simulink model "GridTiedInverterPortedV3"  (R2025a)
settings: Solver=ode23t  StartTime=0.0  StopTime=0.45  FixedStep=Ts  RelTol=1e-3  EnableMultiTasking=on
PreLoadFcn:
  | GridTiedInverterData;
values from neighbouring files (symbols this model uses):
  Ki_vd = 850    [GridTiedInverterData.m]
  Ki_vq = 850    [GridTiedInverterData.m]
  Kp_vd = 0.36    [GridTiedInverterData.m]
  Kp_vq = 0.36    [GridTiedInverterData.m]
  Ts = 1e-6    (= 1e-06)    [GridTiedInverterData.m]
libraries: nesl_utility x20, fl_lib x15, ee_lib x10, eeTransforms x2, slpidlib x2, eePwmGeneratorTwoLevel x1, eeSinusoidalMeasurement x1
CloseFcn:
  | try,close(h1_GridTiedInverter),end
  | clear h1_GridTiedInverter
  | 
  | 
  | clear simlog_GridTiedInverter
  | clear logsout_GridTiedInverter
  | 
  | clear Ts fsw Kp_vd Ki_vd Kp_vq Ki_vq
Description:
  | Three-Phase Grid-Tied Inverter
settings Model: ExtModeTrigDuration=100  Creator=The MathWorks, Inc.  LastModifiedBy=matthiasmees
settings SolverCC: AlgebraicLoopSolver=TrustRegion  MaxZcPerStep=1.0
settings DataIOCC: SaveFormat=StructureWithTime  SaveOutput=off  SaveTime=off  ReturnWorkspaceOutputs=off  SignalLoggingName=logsout_GridTiedInverter
settings OptimizationCC: ReuseModelBlockBuffer=off  ExpressionDepthLimit=2147483647.0  LifeSpan=inf
settings DebuggingCC: UnconnectedInputMsg=warning  UnconnectedOutputMsg=warning  UnconnectedLineMsg=warning  AllowSymbolicDim=off  StateNameClashWarn=warning  SFUnexpectedBacktrackingDiag=warning  SFNoUnconditionalDefaultTransitionDiag=warning  SFExecutionAtInitializationDiag=none  ArithmeticOperatorsInVariantConditions=warning
settings HardwareCC: ProdBitPerPointer=32.0  ProdBitPerSizeT=32.0  ProdBitPerPtrDiffT=32.0  ProdLargestAtomicFloat=None  ProdIntDivRoundTo=Undefined  ProdEndianess=Unspecified  ProdWordSize=32.0  ProdHWDeviceType=32-bit Generic
settings ModelReferenceCC: EnableRefExpFcnMdlSchedulingChecks=on  PropagateSignalLabelsOutOfModel=off
settings SFSimCC: SimUseLocalCustomCode=off  CustomCodeUndefinedFunction=UseInterfaceOnly
settings RTWCC: RTWUseLocalCustomCode=off  GPUComputeCapability=3.5  DLArmComputeVersion=19.05
settings CodeAppCC: StateflowObjectComments=on
settings GRTTargetCC: TargetLangStandard=C89/C90 (ANSI)  CombineOutputUpdateFcns=off  GRTInterface=on
settings ConfigComp: CovMetricSettings=dw  CovSaveCumulativeToWorkspaceVar=on  CovSaveSingleToWorkspaceVar=on  CovExternalEMLEnable=off
settings SimscapeCC: SimscapeNormalizeSystem=off  SimscapeLogType=all  SimscapeLogName=simlog_GridTiedInverter  SimscapeLogLimitData=off

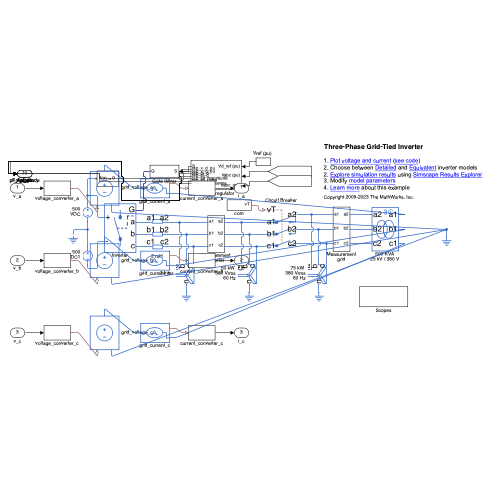
[thumbnail: Simulink's stored preview of the top-level diagram]
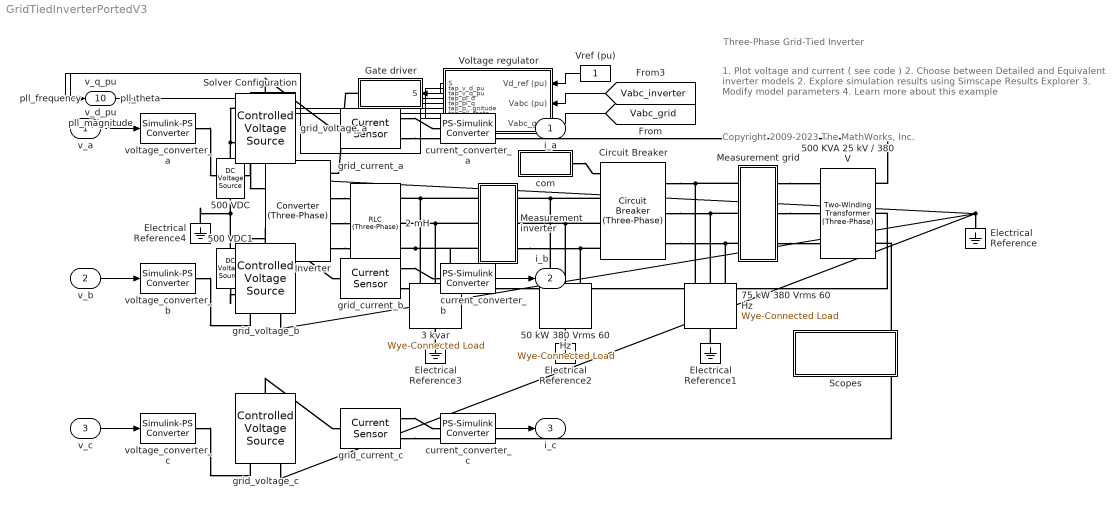
== system GridTiedInverterPortedV3 ==
  note: Three-Phase Grid-Tied Inverter
  note: 1. Plot voltage and current ( see code )
      | 2. Choose between Detailed and Equivalent inverter models
      | 2. Explore simulation results using Simscape Results Explorer
      | 3. Modify model parameters
      | 4. Learn more about this example
  note: Copyright 2009-2023 The MathWorks, Inc.
  v_a : Inport
  v_b : Inport  Port=2
  v_c : Inport  Port=3
  2 mH : ee_lib/Passive/RLC Assemblies/RLC (Three-Phase)  port_option=ee.enum.threePhasePort.expanded  component_structure=ee.enum.rlc.structure.SeriesRL  R=0.02 Ohm  L=0.002 H  C=1 F  R_parasitic=1e-6 Ohm  G_parasitic=1e-6 1/Ohm  IL_specify=on  IL_priority=High  IL=[0, 0, 0] A  IL_nominal_specify=off  IL_nominal_value=1  IL_nominal_unit=A  VC_specify=on  VC_priority=High  VC=[0, 0, 0] V  VC_nominal_specify=off  VC_nominal_value=1  VC_nominal_unit=V
      settings: InternalSimscapePortConfiguration="{\"Bottom\":[],\"Left\":[{\"id\":\"a1\",\"label\":\"a1\",\"type\":\"foundation.electrical.electrical\"},{\"id\":\"b1\",\"label\":\"b1\",\"type\":\"foundation.electrical.electrical\"},{\"id\":\"c1\",\"label\":\"c1\",\"type\":\"foundation.electrical.electrical\"}],\"Right\":[{\"id\":\"a2\",\"label\":\"a2\",\"type\":\"foundation.electrical.electrical\"},{\"id\":\"b2\",\"label\":\"b2\",\"type\":\"foundation.electrical.electrical\"},{\"id\":\"c2\",\"label\":\"c2\",\"type\":\"foundation.electrical.electrical\"}],\"Top\":[]}"
  3 kvar : ee_lib/Passive/RLC Assemblies/Wye-Connected Load  port_option=ee.enum.threePhasePort.expanded  parameterization=ee.enum.rlc.parameterization.ratedpower  component_structure=ee.enum.rlc.structure.C  component_structure_PQ=ee.enum.rlc.structure.C  R=1 Ohm  L=0.001 H  C=1e-6 F  VRated=380 V  FRated=60 Hz  P=0 W  Qpos=0 V*A  Qneg=-3000 V*A  R_parasitic=1e-6 Ohm  G_parasitic=1e-6 1/Ohm  R_parasitic_PQ=1e-6 Ohm  G_parasitic_PQ=1e-6 1/Ohm  Vmag0=0 V  Vang0=0 deg  Freq0=60 Hz  IL_specify=on  IL_priority=High  IL=[ 0 0 0 ] A  IL_nominal_specify=off  IL_nominal_value=1  IL_nominal_unit=A  VC_specify=on  VC_priority=High  VC=[ 0 0 0 ] V  VC_nominal_specify=off  VC_nominal_value=1  VC_nominal_unit=V
      settings: InternalSimscapePortConfiguration="{\"Bottom\":[],\"Left\":[{\"id\":\"a\",\"label\":\"a\",\"type\":\"foundation.electrical.electrical\"},{\"id\":\"b\",\"label\":\"b\",\"type\":\"foundation.electrical.electrical\"},{\"id\":\"c\",\"label\":\"c\",\"type\":\"foundation.electrical.electrical\"}],\"Right\":[{\"id\":\"n\",\"label\":\"n\",\"type\":\"foundation.electrical.electrical\"}],\"Top\":[]}"
  50 kW 380 Vrms 60 Hz : ee_lib/Passive/RLC Assemblies/Wye-Connected Load  port_option=ee.enum.threePhasePort.expanded  parameterization=2  component_structure=1  component_structure_PQ=ee.enum.rlc.structure.R  R=1 Ohm  L=0.001 H  C=1e-6 F  VRated=380 V  FRated=60 Hz  P=50000 W  Qpos=0 V*A  Qneg=-3000 V*A  R_parasitic=1e-6 Ohm  G_parasitic=1e-6 1/Ohm  R_parasitic_PQ=1e-6 Ohm  G_parasitic_PQ=1e-6 1/Ohm  Vmag0=380 V  Vang0=0 deg  Freq0=60 Hz  IL_specify=on  IL_priority=High  IL=[ 0 0 0 ] A  IL_nominal_specify=off  IL_nominal_value=1  IL_nominal_unit=A  VC_specify=on  VC_priority=High  VC=[ 0 0 0 ] V  VC_nominal_specify=off  VC_nominal_value=1  VC_nominal_unit=V
      settings: InternalSimscapePortConfiguration="{\"Bottom\":[],\"Left\":[{\"id\":\"a\",\"label\":\"a\",\"type\":\"foundation.electrical.electrical\"},{\"id\":\"b\",\"label\":\"b\",\"type\":\"foundation.electrical.electrical\"},{\"id\":\"c\",\"label\":\"c\",\"type\":\"foundation.electrical.electrical\"}],\"Right\":[{\"id\":\"n\",\"label\":\"n\",\"type\":\"foundation.electrical.electrical\"}],\"Top\":[]}"
  500 VDC : fl_lib/Electrical/Electrical Sources/DC Voltage Source  v0=500 V
  500 VDC1 : fl_lib/Electrical/Electrical Sources/DC Voltage Source  v0=500 V
  500 KVA 25 kV / 380 V : ee_lib/Passive/Transformers/Two-Winding Transformer (Three-Phase)  SRated=500000 V*A  FRated=60 Hz  Winding1Connection=ee.enum.windingconnection.Y  VRated1=25000 V  Winding2Connection=ee.enum.windingconnection.delta1  VRated2=380 V  CoreType=ee.enum.coretype.fivelimb  pu_Rw1=0.0020  pu_Rw2=0.0020  leakage_reactance_option=ee.enum.transformer_leakage.include  pu_Xl1=0.0800  pu_Xl2=0.0800  magnetizing_resistance_option=ee.enum.transformer_magnetizingResistance.include  pu_Rm=500  magnetizing_reactance_option=ee.enum.transformer_magnetizingReactance.include  saturation_option=ee.enum.transformer_saturation.exclude  pu_Xm=500  current_data=[0, .002, 1, 2]  magnetic_flux_data=[0, 1.2, 1.5, 1.51]  pu_X0=0.5  i1_specify=off  i1_priority=None  i1=[ 0 0 0 ] A  i1_nominal_specify=off  i1_nominal_value=1  i1_nominal_unit=A  i2_specify=off  i2_priority=None  i2=[ 0 0 0 ] A  i2_nominal_specify=off  i2_nominal_value=1  i2_nominal_unit=A  phi_specify=on  phi_priority=None  phi=[0, 0, 0]  phi_nominal_specify=off  phi_nominal_value=1  phi_nominal_unit=1  power_dissipated_specify=off  power_dissipated_priority=None  power_dissipated=0 W  power_dissipated_nominal_specify=off  power_dissipated_nominal_value=1  power_dissipated_nominal_unit=W
      settings: InternalSimscapePortConfiguration="{\"Bottom\":[],\"Left\":[{\"id\":\"a1\",\"label\":\"a1\",\"type\":\"foundation.electrical.electrical\"},{\"id\":\"b1\",\"label\":\"b1\",\"type\":\"foundation.electrical.electrical\"},{\"id\":\"c1\",\"label\":\"c1\",\"type\":\"foundation.electrical.electrical\"}],\"Right\":[{\"id\":\"a2\",\"label\":\"a2\",\"type\":\"foundation.electrical.electrical\"},{\"id\":\"b2\",\"label\":\"b2\",\"type\":\"foundation.electrical.electrical\"},{\"id\":\"c2\",\"label\":\"c2\",\"type\":\"foundation.electrical.electrical\"}],\"Top\":[]}"
  75 kW 380 Vrms 60 Hz : ee_lib/Passive/RLC Assemblies/Wye-Connected Load  port_option=ee.enum.threePhasePort.expanded  parameterization=2  component_structure=1  component_structure_PQ=ee.enum.rlc.structure.R  R=1 Ohm  L=0.001 H  C=1e-6 F  VRated=380 V  FRated=60 Hz  P=75000 W  Qpos=0 V*A  Qneg=-3000 V*A  R_parasitic=1e-6 Ohm  G_parasitic=1e-6 1/Ohm  R_parasitic_PQ=1e-6 Ohm  G_parasitic_PQ=1e-6 1/Ohm  Vmag0=380 V  Vang0=0 deg  Freq0=60 Hz  IL_specify=on  IL_priority=High  IL=[ 0 0 0 ] A  IL_nominal_specify=off  IL_nominal_value=1  IL_nominal_unit=A  VC_specify=on  VC_priority=High  VC=[ 0 0 0 ] V  VC_nominal_specify=off  VC_nominal_value=1  VC_nominal_unit=V
      settings: InternalSimscapePortConfiguration="{\"Bottom\":[],\"Left\":[{\"id\":\"a\",\"label\":\"a\",\"type\":\"foundation.electrical.electrical\"},{\"id\":\"b\",\"label\":\"b\",\"type\":\"foundation.electrical.electrical\"},{\"id\":\"c\",\"label\":\"c\",\"type\":\"foundation.electrical.electrical\"}],\"Right\":[{\"id\":\"n\",\"label\":\"n\",\"type\":\"foundation.electrical.electrical\"}],\"Top\":[]}"
  Circuit Breaker : ee_lib/Switches & Breakers/Circuit Breaker (Three-Phase)  R_closed=0.001 Ohm  G_open=1e-6 1/Ohm  threshold=0.5 V  breaker_behavior=ee.enum.switches.breakerBehavior.zeroCrossingEnable
      settings: InternalSimscapePortConfiguration="{\"Bottom\":[],\"Left\":[{\"id\":\"vT\",\"label\":\"vT\",\"type\":\"input\"},{\"id\":\"a1\",\"label\":\"a1\",\"type\":\"foundation.electrical.electrical\"},{\"id\":\"b1\",\"label\":\"b1\",\"type\":\"foundation.electrical.electrical\"},{\"id\":\"c1\",\"label\":\"c1\",\"type\":\"foundation.electrical.electrical\"}],\"Right\":[{\"id\":\"a2\",\"label\":\"a2\",\"type\":\"foundation.electrical.electrical\"},{\"id\":\"b2\",\"label\":\"b2\",\"type\":\"foundation.electrical.electrical\"},{\"id\":\"c2\",\"label\":\"c2\",\"type\":\"foundation.electrical.electrical\"}],\"Top\":[]}"
  Electrical Reference{,1..4} (5 alike) : fl_lib/Electrical/Electrical Elements/Electrical Reference
  Gate driver : Subsystem
  Inverter : ee_lib/Semiconductors & Converters/Converters/Converter (Three-Phase)  port_option=ee.enum.threePhasePort.expanded  fidelity_option=ee.enum.converters.fidelity.detailed  device_type=ee.enum.converters.switchingdevice.igbt  showThermalPort=false  K=0  Vth=0.5 V  Vgt=0.5 V  Vgt_off=0.1 V  Ih=0.1 A  Vf=1e-6 V  Ron=1e-3 Ohm  Rds=0.001 Ohm  Goff=2e-4 1/Ohm  Eon_scalar=22.86e-3 J  Eoff_scalar=17.14e-3 J  Eoff_natural_commutation=10e-3 J  Voff=300 V  Iout_scalar=600 A  onCurrentMeasDelay=0 s  useCurrentFromPreviousCycle=false  useVoltageFromPreviousCycle=false  diode_param=ee.enum.converters.protectiondiode.nodynamics  diode_Vf=1e-6 V  diode_Ron=1e-3 Ohm  diode_Goff=2e-4 1/Ohm  diode_C=50 nF  diode_iRM=-235 A  diode_iF=300 A  diode_idot=-50 A/us  diode_trr_param=ee.enum.converters.diodetrr.trr_factor  diode_trr_factor=3  diode_trr=15 us  diode_Qrr=1.5e+3 s*uA  diode_rec_loss_model=ee.enum.diode.reverseRecoveryModel.fixed  diode_ErecVal=0 J  diode_scaleWithIandV=false  diode_ErecMat=zeros(2, 3) J  diode_TjrecVec=[298.15, 398.15] K  diode_IfrecVec=[.1, 1, 10] A  diode_IrecVal=10 A  diode_VrecVal=10 V  diode_tFilter=1 / 1000 / 100 s  thermal_network_parameterization=ee.enum.thermalNetworkTopology.external  Rth=[.08, .5] K/W  Rth_Cauer=[.08, .1, .5] K/W  Rth_Foster=[.08, .14, .22, .16] K/W  thermal_mass_parameterization=ee.enum.thermalNetwork.timeconstant  thermal_mass=[.01, .5] J/K  thermal_mass_Cauer=[.01, .1, .5] J/K  thermal_mass_Foster=[.001, .005, .05, .5] J/K  thermal_time_constant=[.001, .2] s  thermal_time_constant_Cauer=[.001, .1, .2] s  thermal_time_constant_Foster=[7e-05, .0007, .01, .08] s  thermal_mass_initial_temperatures=[25, 25] degC  thermal_mass_initial_temperatures_Cauer=[25, 25, 25] degC  junction_thermal_mass=0.01 J/K  Tvec_initial_Foster=[25, 25, 25, 25] degC  snubber_type=ee.enum.converters.snubber.exclude  Cs=1e-7 F  Rs=0.1 Ohm  Vce_loss=[0, 150, 300] V
      settings: InternalSimscapePortConfiguration="{\"Bottom\":[],\"Left\":[{\"id\":\"G\",\"label\":\"G\",\"type\":\"foundation.electrical.twelve_phase\"},{\"id\":\"a\",\"label\":\"a\",\"type\":\"foundation.electrical.electrical\"},{\"id\":\"b\",\"label\":\"b\",\"type\":\"foundation.electrical.electrical\"},{\"id\":\"c\",\"label\":\"c\",\"type\":\"foundation.electrical.electrical\"}],\"Right\":[{\"id\":\"p\",\"label\":\"+\",\"type\":\"foundation.electrical.electrical\"},{\"id\":\"n\",\"label\":\"-\",\"type\":\"foundation.electrical.electrical\"}],\"Top\":[]}"
  Measurement grid : Subsystem
  Measurement inverter : Subsystem
  Scopes : Subsystem
  Solver Configuration : nesl_utility/Solver Configuration  PhysicalDomain=network_engine_domain  SubClassName=solver  LeftPortType=input  RightPortType=generic  Tones=[]  Harmonics=[]  SimulateNoise=off  Profile=off  UseLocalSampling=off  EnableSwitchedLinearOptims=on  FrequencyDomain=off  UseCCode=off  RelTol=0.001  AbsTol=1e-06  MinStep=1e-09  ToWorkspace=off  RevertToSquareIcSolve=off  NumHomotopyIterations=100  PhasorMode=off  PhasorModeNumHarmonics=1  ConsistencySolver=NEWTON_FTOL  IndexReductionMethod=DerivativeReplacement  DoDC=off  ResidualTolerance=1e-09  ConsistencyTolSource=GLOBAL  ConsistencyAbsTol=0.001  ConsistencyRelTol=0.001  ConsistencyTolFactor=0.001  UseLocalSolver=off  LocalSolverChoice=NE_BACKWARD_EULER_ADVANCER  ResolveIndetEquations=on  FunctionEvalNumThread=1  LocalSolverSampleTime=Ts  DoFixedCost=off  MaxNonlinIter=3  MaxModeIter=2  ComputeImpulses=off  ImpulseIterations=1  LinearAlgebra=auto  LinearAlgebraNumThread=0  EquationFormulation=NE_TIME_EF  DelaysMemoryBudget=1024  AutomaticFiltering=on  FilteringTimeConstant=0.001  PartitionStorageMethod=AS_NEEDED  PartitionMemoryBudget=1024  PartitionMethod=FAST  MultibodyUseLocalSolver=off  MultibodyLocalSolverChoice=ODE1  MultibodyLocalSolverSampleTime=0.001
  Voltage regulator : Subsystem
  "Vref (pu) " : Constant
  com : Subsystem
  current_converter_a : nesl_utility/PS-Simulink Converter  PhysicalDomain=network_engine_domain  SubClassName=ps_output  LeftPortType=input  RightPortType=output  PseudoPeriodic=off  Frequencies=[]  VectorFormat=inherit  Unit=A  AffineConversion=off
  current_converter_b : nesl_utility/PS-Simulink Converter  PhysicalDomain=network_engine_domain  SubClassName=ps_output  LeftPortType=input  RightPortType=output  PseudoPeriodic=off  Frequencies=[]  VectorFormat=inherit  Unit=A  AffineConversion=off
  current_converter_c : nesl_utility/PS-Simulink Converter  PhysicalDomain=network_engine_domain  SubClassName=ps_output  LeftPortType=input  RightPortType=output  PseudoPeriodic=off  Frequencies=[]  VectorFormat=inherit  Unit=A  AffineConversion=off
  grid_current_a : fl_lib/Electrical/Electrical Sensors/Current Sensor
  grid_current_b : fl_lib/Electrical/Electrical Sensors/Current Sensor
  grid_current_c : fl_lib/Electrical/Electrical Sensors/Current Sensor
  grid_voltage_a : fl_lib/Electrical/Electrical Sources/Controlled Voltage Source
  grid_voltage_b : fl_lib/Electrical/Electrical Sources/Controlled Voltage Source
  grid_voltage_c : fl_lib/Electrical/Electrical Sources/Controlled Voltage Source
  voltage_converter_a : nesl_utility/Simulink-PS Converter  PhysicalDomain=network_engine_domain  SubClassName=ps_input  LeftPortType=input  RightPortType=output  PseudoPeriodic=off  Frequencies=[]  NoiseDistribution=none  NoiseParameters=[]  Unit=V  AffineConversion=off  FilteringAndDerivatives=provide  SimscapeFilterOrder=1  InputFilterTimeConstant=0.001  UdotUserProvided=0
  voltage_converter_b : nesl_utility/Simulink-PS Converter  PhysicalDomain=network_engine_domain  SubClassName=ps_input  LeftPortType=input  RightPortType=output  PseudoPeriodic=off  Frequencies=[]  NoiseDistribution=none  NoiseParameters=[]  Unit=V  AffineConversion=off  FilteringAndDerivatives=provide  SimscapeFilterOrder=1  InputFilterTimeConstant=0.001  UdotUserProvided=0
  voltage_converter_c : nesl_utility/Simulink-PS Converter  PhysicalDomain=network_engine_domain  SubClassName=ps_input  LeftPortType=input  RightPortType=output  PseudoPeriodic=off  Frequencies=[]  NoiseDistribution=none  NoiseParameters=[]  Unit=V  AffineConversion=off  FilteringAndDerivatives=provide  SimscapeFilterOrder=1  InputFilterTimeConstant=0.001  UdotUserProvided=0
  i_a : Outport
  i_b : Outport  Port=2
  i_c : Outport  Port=3
  v_d_pu : Outport  Port=4
  v_q_pu : Outport  Port=5
  pi_d : Outport  Port=6
  pi_q : Outport  Port=7
  pll_frequency : Outport  Port=8
  pll_theta : Outport  Port=9
  pll_magnitude : Outport  Port=10
  wires:
  [Vabc_grid] -> Voltage regulator/3(Vabc_grid)
  "Vref (pu) "/1 -> Voltage regulator/1(Vd_ref (pu))
  [Vabc_inverter] -> Voltage regulator/2(Vabc (pu))
  Voltage regulator/1(S) -> Gate driver/1(S)
  v_a/1 -> voltage_converter_a/1
  current_converter_a/1 -> i_a/1
  v_b/1 -> voltage_converter_b/1
  current_converter_b/1 -> i_b/1
  v_c/1 -> voltage_converter_c/1
  current_converter_c/1 -> i_c/1
  Voltage regulator/2(tap_v_d_pu) -> v_d_pu/1
  Voltage regulator/3(tap_v_q_pu) -> v_q_pu/1
  Voltage regulator/4(tap_pi_d) -> pi_d/1
  Voltage regulator/5(tap_pi_q) -> pi_q/1
  Voltage regulator/6(tap_pll_magnitude) -> pll_frequency/1
  Voltage regulator/7(tap_pll_theta) -> pll_theta/1
  Voltage regulator/8(tap_pll_frequency) -> pll_magnitude/1
  connections:
  75 kW 380 Vrms 60 Hz/LConn1 -- Measurement grid/LConn1 -- Circuit Breaker/RConn1
  3 kvar/LConn2 -- Measurement inverter/LConn2 -- 2 mH/RConn2
  Circuit Breaker/LConn2 -- 50 kW 380 Vrms 60 Hz/LConn1 -- Measurement inverter/RConn1
  Circuit Breaker/RConn2 -- Measurement grid/LConn2 -- 75 kW 380 Vrms 60 Hz/LConn2
  Measurement grid/RConn3 -- 500 KVA 25 kV / 380 V/RConn3
  500 VDC/LConn1 -- Solver Configuration/RConn1 -- Inverter/RConn1
  Circuit Breaker/RConn3 -- Measurement grid/LConn3 -- 75 kW 380 Vrms 60 Hz/LConn3
  50 kW 380 Vrms 60 Hz/LConn3 -- Circuit Breaker/LConn4 -- Measurement inverter/RConn3
  Inverter/LConn4 -- 2 mH/LConn3
  Electrical Reference1/LConn1 -- 75 kW 380 Vrms 60 Hz/RConn1
  Gate driver/RConn1 -- Inverter/LConn1
  Electrical Reference2/LConn1 -- 50 kW 380 Vrms 60 Hz/RConn1
  com/RConn1 -- Circuit Breaker/LConn1
  Electrical Reference3/LConn1 -- 3 kvar/RConn1
  Inverter/LConn2 -- 2 mH/LConn1
  Inverter/LConn3 -- 2 mH/LConn2
  3 kvar/LConn1 -- 2 mH/RConn1 -- Measurement inverter/LConn1
  2 mH/RConn3 -- Measurement inverter/LConn3 -- 3 kvar/LConn3
  Circuit Breaker/LConn3 -- 50 kW 380 Vrms 60 Hz/LConn2 -- Measurement inverter/RConn2
  Measurement grid/RConn1 -- 500 KVA 25 kV / 380 V/RConn1
  Measurement grid/RConn2 -- 500 KVA 25 kV / 380 V/RConn2
  500 VDC1/RConn1 -- Inverter/RConn2
  500 VDC1/LConn1 -- Electrical Reference4/LConn1 -- 500 VDC/RConn1
  voltage_converter_a/RConn1 -- grid_voltage_a/RConn1
  grid_voltage_a/LConn1 -- grid_current_a/LConn1
  grid_current_a/RConn2 -- 500 KVA 25 kV / 380 V/LConn1
  grid_current_a/RConn1 -- current_converter_a/LConn1
  voltage_converter_b/RConn1 -- grid_voltage_b/RConn1
  grid_voltage_b/LConn1 -- grid_current_b/LConn1
  grid_current_b/RConn2 -- 500 KVA 25 kV / 380 V/LConn2
  grid_current_b/RConn1 -- current_converter_b/LConn1
  voltage_converter_c/RConn1 -- grid_voltage_c/RConn1
  grid_voltage_c/LConn1 -- grid_current_c/LConn1
  grid_current_c/RConn2 -- 500 KVA 25 kV / 380 V/LConn3
  grid_current_c/RConn1 -- current_converter_c/LConn1
  grid_voltage_a/RConn2 -- grid_voltage_b/RConn2 -- Electrical Reference/LConn1 -- grid_voltage_c/RConn2

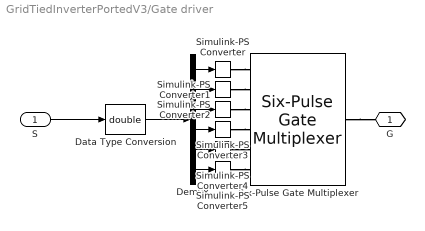
== system GridTiedInverterPortedV3/Gate driver ==
  S : Inport
  Data Type Conversion : DataTypeConversion  OutDataTypeStr=double  SaturateOnIntegerOverflow=off  RndMeth=Floor
  Demux : Demux  Outputs=6
  Simulink-PS Converter{,1..5} (6 alike) : nesl_utility/Simulink-PS Converter  PhysicalDomain=network_engine_domain  SubClassName=ps_input  LeftPortType=input  RightPortType=output  PseudoPeriodic=off  Frequencies=[]  NoiseDistribution=none  NoiseParameters=[]  Unit=1  AffineConversion=off  FilteringAndDerivatives=provide  SimscapeFilterOrder=1  InputFilterTimeConstant=0.001  UdotUserProvided=0
  Six-Pulse Gate Multiplexer : ee_lib/Semiconductors & Converters/Converters/Six-Pulse Gate Multiplexer  port_option=ee.enum.controlport.ps
  G : PMIOPort  Side=Right
  wires:
  Demux/5 -> Simulink-PS Converter4/1
  Demux/3 -> Simulink-PS Converter2/1
  Data Type Conversion/1 -> Demux/1
  Demux/4 -> Simulink-PS Converter3/1
  Demux/6 -> Simulink-PS Converter5/1
  Demux/2 -> Simulink-PS Converter1/1
  Demux/1 -> Simulink-PS Converter/1
  S/1 -> Data Type Conversion/1
  connections:
  Simulink-PS Converter4/RConn1 -- Six-Pulse Gate Multiplexer/LConn5
  Simulink-PS Converter2/RConn1 -- Six-Pulse Gate Multiplexer/LConn3
  Simulink-PS Converter/RConn1 -- Six-Pulse Gate Multiplexer/LConn1
  Simulink-PS Converter5/RConn1 -- Six-Pulse Gate Multiplexer/LConn6
  Simulink-PS Converter1/RConn1 -- Six-Pulse Gate Multiplexer/LConn2
  Simulink-PS Converter3/RConn1 -- Six-Pulse Gate Multiplexer/LConn4
  Six-Pulse Gate Multiplexer/RConn1 -- G/RConn1

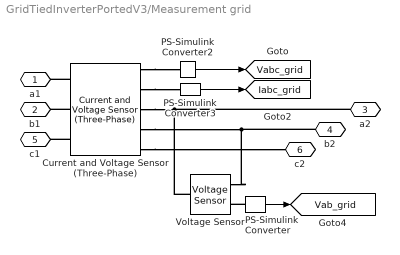
== system GridTiedInverterPortedV3/Measurement grid ==
  Current and Voltage Sensor (Three-Phase) : ee_lib/Sensors & Transducers/Current and Voltage Sensor (Three-Phase)  vMeasurementType=2  outputUnit=ee.enum.unit.pu  SRated=250000 V*A  VRated=380 V  I_specify=off  I_priority=None  I=[ 0 0 0 ] A  I_nominal_specify=off  I_nominal_value=1  I_nominal_unit=A  V_specify=off  V_priority=None  V=[ 0 0 0 ] V  V_nominal_specify=off  V_nominal_value=1  V_nominal_unit=V
      settings: InternalSimscapePortConfiguration="{\"Bottom\":[],\"Left\":[{\"id\":\"a1\",\"label\":\"a1\",\"type\":\"foundation.electrical.electrical\"},{\"id\":\"b1\",\"label\":\"b1\",\"type\":\"foundation.electrical.electrical\"},{\"id\":\"c1\",\"label\":\"c1\",\"type\":\"foundation.electrical.electrical\"}],\"Right\":[{\"id\":\"V_output\",\"label\":\"V\",\"type\":\"output\"},{\"id\":\"I_output\",\"label\":\"I\",\"type\":\"output\"},{\"id\":\"a2\",\"label\":\"a2\",\"type\":\"foundation.electrical.electrical\"},{\"id\":\"b2\",\"label\":\"b2\",\"type\":\"foundation.electrical.electrical\"},{\"id\":\"c2\",\"label\":\"c2\",\"type\":\"foundation.electrical.electrical\"}],\"Top\":[]}"
  PS-Simulink Converter : nesl_utility/PS-Simulink Converter  PhysicalDomain=network_engine_domain  SubClassName=ps_output  LeftPortType=input  RightPortType=output  PseudoPeriodic=off  Frequencies=[]  VectorFormat=1-D array  Unit=V  AffineConversion=off
  PS-Simulink Converter2 : nesl_utility/PS-Simulink Converter  PhysicalDomain=network_engine_domain  SubClassName=ps_output  LeftPortType=input  RightPortType=output  PseudoPeriodic=off  Frequencies=[]  VectorFormat=1-D array  Unit=1  AffineConversion=off
  PS-Simulink Converter3 : nesl_utility/PS-Simulink Converter  PhysicalDomain=network_engine_domain  SubClassName=ps_output  LeftPortType=input  RightPortType=output  PseudoPeriodic=off  Frequencies=[]  VectorFormat=1-D array  Unit=1  AffineConversion=off
  Voltage Sensor : fl_lib/Electrical/Electrical Sensors/Voltage Sensor
  a1 : PMIOPort  Side=Left
  b1 : PMIOPort  Port=2  Side=Left
  a2 : PMIOPort  Port=3  Side=Right
  b2 : PMIOPort  Port=4  Side=Right
  c1 : PMIOPort  Port=5  Side=Left
  c2 : PMIOPort  Port=6  Side=Right
  tag scope: Iabc_grid=global, Vab_grid=global, Vabc_grid=global
  wires:
  PS-Simulink Converter2/1 -> [Vabc_grid]
  PS-Simulink Converter3/1 -> [Iabc_grid]
  PS-Simulink Converter/1 -> [Vab_grid]
  connections:
  b2/RConn1 -- Voltage Sensor/RConn2 -- Current and Voltage Sensor (Three-Phase)/RConn4
  a2/RConn1 -- Voltage Sensor/LConn1 -- Current and Voltage Sensor (Three-Phase)/RConn3
  Current and Voltage Sensor (Three-Phase)/RConn5 -- c2/RConn1
  Current and Voltage Sensor (Three-Phase)/LConn2 -- b1/RConn1
  Current and Voltage Sensor (Three-Phase)/LConn3 -- c1/RConn1
  Current and Voltage Sensor (Three-Phase)/LConn1 -- a1/RConn1
  Current and Voltage Sensor (Three-Phase)/RConn1 -- PS-Simulink Converter2/LConn1
  Current and Voltage Sensor (Three-Phase)/RConn2 -- PS-Simulink Converter3/LConn1
  PS-Simulink Converter/LConn1 -- Voltage Sensor/RConn1

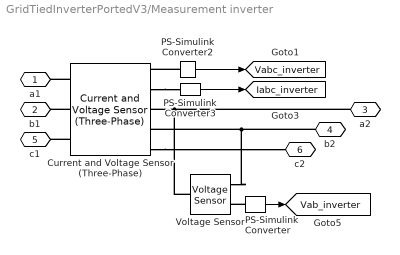
== system GridTiedInverterPortedV3/Measurement inverter ==
  Current and Voltage Sensor (Three-Phase) : ee_lib/Sensors & Transducers/Current and Voltage Sensor (Three-Phase)  vMeasurementType=2  outputUnit=1  SRated=150000 V*A  VRated=380 V  I_specify=off  I_priority=None  I=[ 0 0 0 ] A  I_nominal_specify=off  I_nominal_value=1  I_nominal_unit=A  V_specify=off  V_priority=None  V=[ 0 0 0 ] V  V_nominal_specify=off  V_nominal_value=1  V_nominal_unit=V
      settings: InternalSimscapePortConfiguration="{\"Bottom\":[],\"Left\":[{\"id\":\"a1\",\"label\":\"a1\",\"type\":\"foundation.electrical.electrical\"},{\"id\":\"b1\",\"label\":\"b1\",\"type\":\"foundation.electrical.electrical\"},{\"id\":\"c1\",\"label\":\"c1\",\"type\":\"foundation.electrical.electrical\"}],\"Right\":[{\"id\":\"V_output\",\"label\":\"V\",\"type\":\"output\"},{\"id\":\"I_output\",\"label\":\"I\",\"type\":\"output\"},{\"id\":\"a2\",\"label\":\"a2\",\"type\":\"foundation.electrical.electrical\"},{\"id\":\"b2\",\"label\":\"b2\",\"type\":\"foundation.electrical.electrical\"},{\"id\":\"c2\",\"label\":\"c2\",\"type\":\"foundation.electrical.electrical\"}],\"Top\":[]}"
  PS-Simulink Converter : nesl_utility/PS-Simulink Converter  PhysicalDomain=network_engine_domain  SubClassName=ps_output  LeftPortType=input  RightPortType=output  PseudoPeriodic=off  Frequencies=[]  VectorFormat=1-D array  Unit=V  AffineConversion=off
  PS-Simulink Converter2 : nesl_utility/PS-Simulink Converter  PhysicalDomain=network_engine_domain  SubClassName=ps_output  LeftPortType=input  RightPortType=output  PseudoPeriodic=off  Frequencies=[]  VectorFormat=1-D array  Unit=1  AffineConversion=off
  PS-Simulink Converter3 : nesl_utility/PS-Simulink Converter  PhysicalDomain=network_engine_domain  SubClassName=ps_output  LeftPortType=input  RightPortType=output  PseudoPeriodic=off  Frequencies=[]  VectorFormat=1-D array  Unit=1  AffineConversion=off
  Voltage Sensor : fl_lib/Electrical/Electrical Sensors/Voltage Sensor
  a1 : PMIOPort  Side=Left
  b1 : PMIOPort  Port=2  Side=Left
  a2 : PMIOPort  Port=3  Side=Right
  b2 : PMIOPort  Port=4  Side=Right
  c1 : PMIOPort  Port=5  Side=Left
  c2 : PMIOPort  Port=6  Side=Right
  tag scope: Iabc_inverter=global, Vab_inverter=global, Vabc_inverter=global
  wires:
  PS-Simulink Converter2/1 -> [Vabc_inverter]
  PS-Simulink Converter3/1 -> [Iabc_inverter]
  PS-Simulink Converter/1 -> [Vab_inverter]
  connections:
  b2/RConn1 -- Voltage Sensor/RConn2 -- Current and Voltage Sensor (Three-Phase)/RConn4
  a2/RConn1 -- Voltage Sensor/LConn1 -- Current and Voltage Sensor (Three-Phase)/RConn3
  Current and Voltage Sensor (Three-Phase)/RConn5 -- c2/RConn1
  Current and Voltage Sensor (Three-Phase)/LConn2 -- b1/RConn1
  Current and Voltage Sensor (Three-Phase)/LConn3 -- c1/RConn1
  Current and Voltage Sensor (Three-Phase)/LConn1 -- a1/RConn1
  PS-Simulink Converter2/LConn1 -- Current and Voltage Sensor (Three-Phase)/RConn1
  Current and Voltage Sensor (Three-Phase)/RConn2 -- PS-Simulink Converter3/LConn1
  PS-Simulink Converter/LConn1 -- Voltage Sensor/RConn1

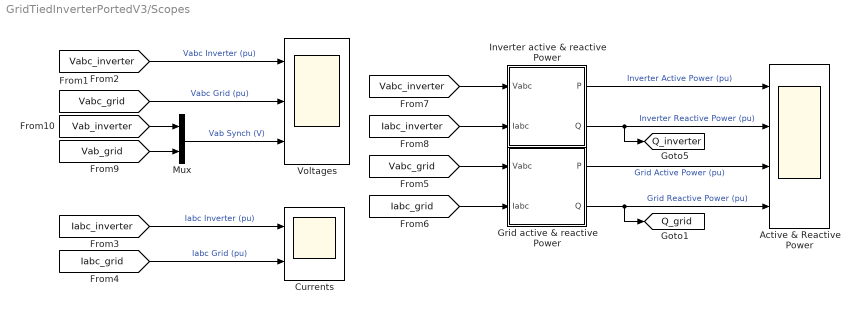
== system GridTiedInverterPortedV3/Scopes ==
  Active & Reactive Power : Scope  NumInputPorts=4
      settings: ActiveDisplayYMinimum=-0.09819  ActiveDisplayYMaximum=0.88371  DataLoggingDecimation=10
  Currents : Scope  NumInputPorts=2
      settings: ActiveDisplayYMinimum=-0.75017  ActiveDisplayYMaximum=0.74928  DataLoggingVariableName=ScopeData2
  Grid active & reactive Power : Subsystem
  "Inverter active & reactive Power " : Subsystem
  Mux : Mux  Inputs=2
  Voltages : Scope  NumInputPorts=3
      settings: ActiveDisplayYMinimum=-1.26809  ActiveDisplayYMaximum=1.26724
  tag scope: Q_grid=global, Q_inverter=global
  wires:
  [Iabc_grid] -> Grid active & reactive Power/2(Iabc)
  "Inverter active & reactive Power "/2(Q) -> Active & Reactive Power/2, [Q_inverter]  "Inverter Reactive Power (pu)"
  [Vab_grid] -> Mux/2
  [Vab_inverter] -> Mux/1
  [Iabc_inverter] -> Currents/1  "Iabc Inverter (pu)"
  Mux/1 -> Voltages/3  "Vab Synch (V)"
  [Vabc_inverter] -> Voltages/1  "Vabc Inverter (pu)"
  [Iabc_inverter] -> "Inverter active & reactive Power "/2(Iabc)
  [Vabc_grid] -> Grid active & reactive Power/1(Vabc)
  [Vabc_inverter] -> "Inverter active & reactive Power "/1(Vabc)
  [Iabc_grid] -> Currents/2  "Iabc Grid (pu)"
  [Vabc_grid] -> Voltages/2  "Vabc Grid (pu)"
  Grid active & reactive Power/2(Q) -> [Q_grid], Active & Reactive Power/4  "Grid Reactive Power (pu)"
  "Inverter active & reactive Power "/1(P) -> Active & Reactive Power/1  "Inverter Active Power (pu)"
  Grid active & reactive Power/1(P) -> Active & Reactive Power/3  "Grid Active Power (pu)"

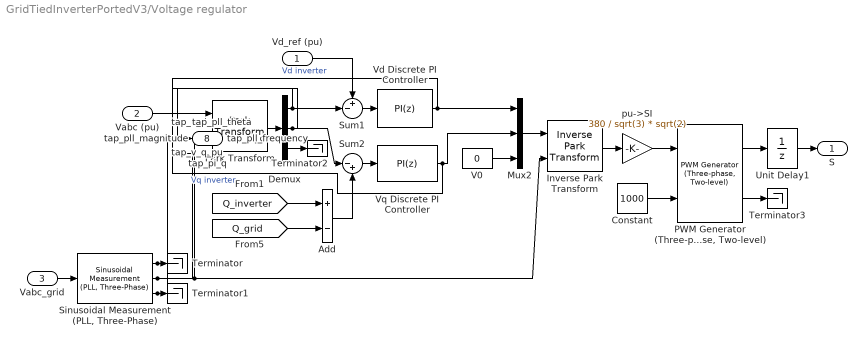
== system GridTiedInverterPortedV3/Voltage regulator ==
  Vd_ref (pu) : Inport
  Vabc (pu) : Inport  Port=2
  Vabc_grid : Inport  Port=3
  Add : Sum  Inputs=+-
  Constant : Constant  Value=1000
  Demux : Demux  Outputs=3
  Inverse Park Transform : eeTransforms/Inverse Park Transform  AxisAlignment=Q-axis  PowerInvariant=off
  Mux2 : Mux  Inputs=3
  "PWM Generator (Three-phase, Two-level)" : eePwmGeneratorTwoLevel/PWM Generator (Three-phase, Two-level)  PWMMode=Continuous PWM (CPWM)  CPWMMode=SPWM: sinusoidal PWM  DPWMMode=60 DPWM: 60 degree discontinuous PWM  fsw=fsw  Ts=Ts
  Park Transform : eeTransforms/Park Transform  AxisAlignment=Q-axis  PowerInvariant=off
  "Sinusoidal Measurement (PLL, Three-Phase)" : eeSinusoidalMeasurement/Sinusoidal Measurement (PLL, Three-Phase)  Kp_LF=150  Ki_LF=150  F0=60  Theta0=0  Ts=Ts
  Sum1 : Sum  Inputs=+-|  InputSameDT=on  SaturateOnIntegerOverflow=on  OutDataTypeStr=Inherit: Same as first input
  Sum2 : Sum  Inputs=|-+  InputSameDT=on  SaturateOnIntegerOverflow=on  OutDataTypeStr=Inherit: Same as first input
  Terminator{,1..3} (4 alike) : Terminator
  Unit Delay1 : UnitDelay  SampleTime=Ts  HasFrameUpgradeWarning=on
  V0 : Constant  Value=0
  Vd Discrete PI Controller : slpidlib/PID Controller  Controller=PI  Form=Parallel  TimeDomain=Discrete-time  UseExternalTs=off  SampleTime=Ts  IntegratorMethod=Forward Euler  FilterMethod=Forward Euler  ControllerParametersSource=internal  P=Kp_vd  I=Ki_vd  UseKiTs=off  D=0  UseExternalDerivativeSource=off  N=100  UseFilter=on  TunerSelectOption=Transfer Function Based (PID Tuner App)  InitialConditionSource=internal  InitialConditionForIntegrator=0  InitialConditionForFilter=0  DifferentiatorICPrevScaledInput=0  ExternalReset=none  TrackingMode=off  Kt=1  LimitOutput=on  SatLimitsSource=internal  UpperSaturationLimit=1  LowerSaturationLimit=0  LinearizeAsGain=on  AntiWindupMode=none  Kb=1  LimitIntegrator=off  UpperIntegratorSaturationLimit=inf  LowerIntegratorSaturationLimit=-inf  POutMin=[]  POutMax=[]  IOutMin=[]  IOutMax=[]  DOutMin=[]  DOutMax=[]  NOutMin=[]  NOutMax=[]  SumOutMin=[]  SumOutMax=[]  SaturationOutMin=[]  SaturationOutMax=[]  PParamMin=[]  PParamMax=[]  IParamMin=[]  IParamMax=[]  DParamMin=[]  DParamMax=[]  NParamMin=[]  NParamMax=[]  KbParamMin=[]  KbParamMax=[]  KtParamMin=[]  KtParamMax=[]  KbOutMin=[]  KbOutMax=[]  KtOutMin=[]  KtOutMax=[]  IntegratorOutMin=[]  IntegratorOutMax=[]  FilterOutMin=[]  FilterOutMax=[]  SumI1OutMin=[]  SumI1OutMax=[]  SumI2OutMin=[]  SumI2OutMax=[]  SumI3OutMin=[]  SumI3OutMax=[]  SumI4OutMin=[]  SumI4OutMax=[]  SumDOutMin=[]  SumDOutMax=[]  DifferentiatorOutMin=[]  DifferentiatorOutMax=[]  FilterDiffOutCoefMin=[]  FilterDiffOutCoefMax=[]  ReciprocalOutMin=[]  ReciprocalOutMax=[]  SumDenOutMin=[]  SumDenOutMax=[]  SumNumOutMin=[]  SumNumOutMax=[]  DivideOutMin=[]  DivideOutMax=[]  UdiffTsProdOutMin=[]  UdiffTsProdOutMax=[]  NTsProdOutMin=[]  NTsProdOutMax=[]  UintegralTsProdOutMin=[]  UintegralTsProdOutMax=[]  UngainTsProdOutMin=[]  UngainTsProdOutMax=[]  ClampingZeroOutDataTypeStr=Inherit: Inherit via back propagation  ClampingZeroOutMin=[]  ClampingZeroOutMax=[]  FilterDenConstantOutDataTypeStr=Inherit: Inherit via back propagation  FilterDenConstantOutMin=[]  FilterDenConstantOutMax=[]  PCopyOutDataTypeStr=Inherit: Inherit via back propagation  PCopyOutMin=[]  PCopyOutMax=[]  NCopyOutDataTypeStr=Inherit: Inherit via back propagation  NCopyOutMin=[]  NCopyOutMax=[]  IntegratorContinuousStateAttributes=''  IntegratorStateMustResolveToSignalObject=off  IntegratorRTWStateStorageClass=Auto  FilterContinuousStateAttributes=''  FilterStateMustResolveToSignalObject=off  FilterRTWStateStorageClass=Auto  ParallelPVariant=InternalParameters  IdealPVariant=Disabled  IVariant=InternalParameters  DVariant=Disabled  IntegratorVariant=Discrete  SatVariant=Enabled  AWVariant=Passthrough  PCopyVariant=Disabled  TRVariant=Disabled  FdbkBlocksVariant=Forward  IdealPFdbkVariant=Disabled  SatFdbkVariant=Disabled  DerivativeFilterVariant=Disabled  NVariant=Disabled  NCopyVariant=Disabled_SignalSpec  FilterICVariant=Disabled  IntegratorICVariant=InternalICs  ExternalResetVariant=Disabled  TRSumVariant=Passthrough  SumFdbkVariant=Disabled  SumVariant=Sum_PI  TsampFilterVariant=InternalTs  TsampNgainVariant=Passthrough  TsampIntegralVariant=Disabled_SignalSpec  ExternalSaturationOutDataTypeStr=Inherit: Same as second input  DerivativeSourceVariant=Disabled  PreIntVariant=InternalPreInt
  Vq Discrete PI Controller : slpidlib/PID Controller  Controller=PI  Form=Parallel  TimeDomain=Discrete-time  UseExternalTs=off  SampleTime=Ts  IntegratorMethod=Forward Euler  FilterMethod=Forward Euler  ControllerParametersSource=internal  P=Kp_vq  I=Ki_vq  UseKiTs=off  D=0  UseExternalDerivativeSource=off  N=100  UseFilter=on  TunerSelectOption=Transfer Function Based (PID Tuner App)  InitialConditionSource=internal  InitialConditionForIntegrator=0  InitialConditionForFilter=0  DifferentiatorICPrevScaledInput=0  ExternalReset=none  TrackingMode=off  Kt=1  LimitOutput=on  SatLimitsSource=internal  UpperSaturationLimit=1  LowerSaturationLimit=0  LinearizeAsGain=on  AntiWindupMode=none  Kb=1  LimitIntegrator=off  UpperIntegratorSaturationLimit=inf  LowerIntegratorSaturationLimit=-inf  POutMin=[]  POutMax=[]  IOutMin=[]  IOutMax=[]  DOutMin=[]  DOutMax=[]  NOutMin=[]  NOutMax=[]  SumOutMin=[]  SumOutMax=[]  SaturationOutMin=[]  SaturationOutMax=[]  PParamMin=[]  PParamMax=[]  IParamMin=[]  IParamMax=[]  DParamMin=[]  DParamMax=[]  NParamMin=[]  NParamMax=[]  KbParamMin=[]  KbParamMax=[]  KtParamMin=[]  KtParamMax=[]  KbOutMin=[]  KbOutMax=[]  KtOutMin=[]  KtOutMax=[]  IntegratorOutMin=[]  IntegratorOutMax=[]  FilterOutMin=[]  FilterOutMax=[]  SumI1OutMin=[]  SumI1OutMax=[]  SumI2OutMin=[]  SumI2OutMax=[]  SumI3OutMin=[]  SumI3OutMax=[]  SumI4OutMin=[]  SumI4OutMax=[]  SumDOutMin=[]  SumDOutMax=[]  DifferentiatorOutMin=[]  DifferentiatorOutMax=[]  FilterDiffOutCoefMin=[]  FilterDiffOutCoefMax=[]  ReciprocalOutMin=[]  ReciprocalOutMax=[]  SumDenOutMin=[]  SumDenOutMax=[]  SumNumOutMin=[]  SumNumOutMax=[]  DivideOutMin=[]  DivideOutMax=[]  UdiffTsProdOutMin=[]  UdiffTsProdOutMax=[]  NTsProdOutMin=[]  NTsProdOutMax=[]  UintegralTsProdOutMin=[]  UintegralTsProdOutMax=[]  UngainTsProdOutMin=[]  UngainTsProdOutMax=[]  ClampingZeroOutDataTypeStr=Inherit: Inherit via back propagation  ClampingZeroOutMin=[]  ClampingZeroOutMax=[]  FilterDenConstantOutDataTypeStr=Inherit: Inherit via back propagation  FilterDenConstantOutMin=[]  FilterDenConstantOutMax=[]  PCopyOutDataTypeStr=Inherit: Inherit via back propagation  PCopyOutMin=[]  PCopyOutMax=[]  NCopyOutDataTypeStr=Inherit: Inherit via back propagation  NCopyOutMin=[]  NCopyOutMax=[]  IntegratorContinuousStateAttributes=''  IntegratorStateMustResolveToSignalObject=off  IntegratorRTWStateStorageClass=Auto  FilterContinuousStateAttributes=''  FilterStateMustResolveToSignalObject=off  FilterRTWStateStorageClass=Auto  ParallelPVariant=InternalParameters  IdealPVariant=Disabled  IVariant=InternalParameters  DVariant=Disabled  IntegratorVariant=Discrete  SatVariant=Enabled  AWVariant=Passthrough  PCopyVariant=Disabled  TRVariant=Disabled  FdbkBlocksVariant=Forward  IdealPFdbkVariant=Disabled  SatFdbkVariant=Disabled  DerivativeFilterVariant=Disabled  NVariant=Disabled  NCopyVariant=Disabled_SignalSpec  FilterICVariant=Disabled  IntegratorICVariant=InternalICs  ExternalResetVariant=Disabled  TRSumVariant=Passthrough  SumFdbkVariant=Disabled  SumVariant=Sum_PI  TsampFilterVariant=InternalTs  TsampNgainVariant=Passthrough  TsampIntegralVariant=Disabled_SignalSpec  ExternalSaturationOutDataTypeStr=Inherit: Same as second input  DerivativeSourceVariant=Disabled  PreIntVariant=InternalPreInt
  pu->SI : Gain  Gain=380 / sqrt(3) * sqrt(2)
  S : Outport
  tap_v_d_pu : Outport  Port=2
  tap_v_q_pu : Outport  Port=3
  tap_pi_d : Outport  Port=4
  tap_pi_q : Outport  Port=5
  tap_pll_magnitude : Outport  Port=6
  tap_pll_theta : Outport  Port=7
  tap_pll_frequency : Outport  Port=8
  wires:
  Vd Discrete PI Controller/1 -> Mux2/1, tap_pi_d/1  "Vd inverter"
  "Sinusoidal Measurement (PLL, Three-Phase)"/2 -> Park Transform/2, Inverse Park Transform/2, tap_pll_theta/1
  Mux2/1 -> Inverse Park Transform/1
  Sum1/1 -> Vd Discrete PI Controller/1
  Vabc (pu)/1 -> Park Transform/1
  Park Transform/1 -> Demux/1
  Sum2/1 -> Vq Discrete PI Controller/1
  Add/1 -> Sum2/2
  Demux/2 -> Sum2/1, tap_v_q_pu/1
  Vq Discrete PI Controller/1 -> Mux2/2, tap_pi_q/1  "Vq inverter"
  V0/1 -> Mux2/3
  Demux/1 -> Sum1/2, tap_v_d_pu/1
  Vd_ref (pu)/1 -> Sum1/1
  Demux/3 -> Terminator2/1
  "PWM Generator (Three-phase, Two-level)"/1 -> Unit Delay1/1
  Unit Delay1/1 -> S/1
  Constant/1 -> "PWM Generator (Three-phase, Two-level)"/2
  Inverse Park Transform/1 -> pu->SI/1
  "PWM Generator (Three-phase, Two-level)"/2 -> Terminator3/1
  "Sinusoidal Measurement (PLL, Three-Phase)"/3 -> Terminator1/1, tap_pll_frequency/1
  "Sinusoidal Measurement (PLL, Three-Phase)"/1 -> Terminator/1, tap_pll_magnitude/1
  Vabc_grid/1 -> "Sinusoidal Measurement (PLL, Three-Phase)"/1
  [Q_grid] -> Add/2
  [Q_inverter] -> Add/1
  pu->SI/1 -> "PWM Generator (Three-phase, Two-level)"/1

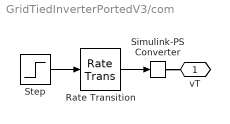
== system GridTiedInverterPortedV3/com ==
  Rate Transition : RateTransition  Integrity=off  OutPortSampleTimeOpt=Inherit
  Simulink-PS Converter : nesl_utility/Simulink-PS Converter  PhysicalDomain=network_engine_domain  SubClassName=ps_input  LeftPortType=input  RightPortType=output  PseudoPeriodic=off  Frequencies=[]  NoiseDistribution=none  NoiseParameters=[]  Unit=1  AffineConversion=off  FilteringAndDerivatives=provide  SimscapeFilterOrder=1  InputFilterTimeConstant=0.001  UdotUserProvided=0
  Step : Step  Time=0.15  Before=1  After=0  SampleTime=0
  vT : PMIOPort  Side=Right
  wires:
  Rate Transition/1 -> Simulink-PS Converter/1
  Step/1 -> Rate Transition/1
  connections:
  Simulink-PS Converter/RConn1 -- vT/RConn1

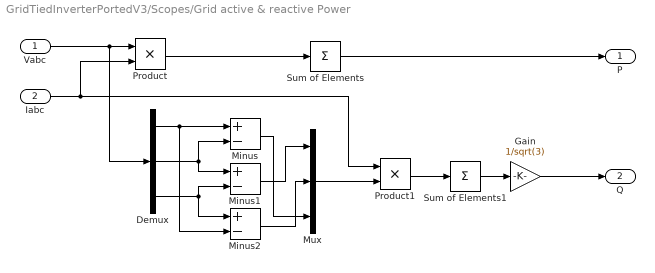
== system GridTiedInverterPortedV3/Scopes/Grid active & reactive Power ==
  Vabc : Inport
  Iabc : Inport  Port=2
  Demux : Demux  Outputs=3
  Gain : Gain  Gain=1/sqrt(3)
  Minus : Sum  Inputs=+-
  Minus1 : Sum  Inputs=+-
  Minus2 : Sum  Inputs=+-
  Mux : Mux  Inputs=3
  Product : Product
  Product1 : Product
  Sum of Elements : Sum  Inputs=+
  Sum of Elements1 : Sum  Inputs=+
  P : Outport  VectorParamsAs1DForOutWhenUnconnected=off
  Q : Outport  Port=2  VectorParamsAs1DForOutWhenUnconnected=off
  wires:
  Minus/1 -> Mux/3
  Minus2/1 -> Mux/2
  Minus1/1 -> Mux/1
  Gain/1 -> Q/1
  Sum of Elements1/1 -> Gain/1
  Product1/1 -> Sum of Elements1/1
  Mux/1 -> Product1/2
  Demux/3 -> Minus1/2, Minus2/1
  Demux/2 -> Minus/2, Minus1/1
  Demux/1 -> Minus/1, Minus2/2
  Sum of Elements/1 -> P/1
  Product/1 -> Sum of Elements/1
  Iabc/1 -> Product/2, Product1/1
  Vabc/1 -> Product/1, Demux/1

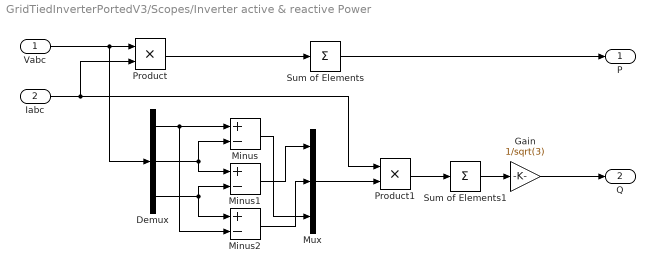
== system GridTiedInverterPortedV3/Scopes/Inverter active & reactive Power  ==
  Vabc : Inport
  Iabc : Inport  Port=2
  Demux : Demux  Outputs=3
  Gain : Gain  Gain=1/sqrt(3)
  Minus : Sum  Inputs=+-
  Minus1 : Sum  Inputs=+-
  Minus2 : Sum  Inputs=+-
  Mux : Mux  Inputs=3
  Product : Product
  Product1 : Product
  Sum of Elements : Sum  Inputs=+
  Sum of Elements1 : Sum  Inputs=+
  P : Outport  VectorParamsAs1DForOutWhenUnconnected=off
  Q : Outport  Port=2  VectorParamsAs1DForOutWhenUnconnected=off
  wires:
  Minus/1 -> Mux/3
  Minus2/1 -> Mux/2
  Minus1/1 -> Mux/1
  Gain/1 -> Q/1
  Sum of Elements1/1 -> Gain/1
  Product1/1 -> Sum of Elements1/1
  Mux/1 -> Product1/2
  Demux/3 -> Minus1/2, Minus2/1
  Demux/2 -> Minus/2, Minus1/1
  Demux/1 -> Minus/1, Minus2/2
  Sum of Elements/1 -> P/1
  Product/1 -> Sum of Elements/1
  Iabc/1 -> Product/2, Product1/1
  Vabc/1 -> Product/1, Demux/1
